simulink model "snap_sys_clk_feng"  (R2019a)
settings: Solver=VariableStepDiscrete  StartTime=0.0  StopTime=10.0  RelTol=1e-3
undefined symbols (not defined in the file): datetime, posixtime
libraries: xbsIndex_r4 x5252, casper_library_misc x69, xps_library x6, casper_library_delays x3
(part 5 of 45)

== system snap_sys_clk_feng/chan_reorder/skip_c_t_transpose ==
  sim_1 : Inport
  convert1_1 : DataTypeConversion  OutDataTypeStr=fixdt('ufix1_En0')  LockScale=on
  convert2_1 : DataTypeConversion  OutDataTypeStr=fixdt('ufix1_En0')  ConvertRealWorld=Stored Integer (SI)  LockScale=on
  gain_1 : Gain
  io_delay : xbsIndex_r4/Delay  rst=off  infoeditControl=Selection of Reset will increase slice count due to use of real FFs and instead of SRLs  en=off  latency=0  reg_retiming=on  dbl_ovrd=off  block_type=delay
  reint1 : xbsIndex_r4/Reinterpret  force_arith_type=on  arith_type=Unsigned  force_bin_pt=on  bin_pt=0  block_type=reinterpret
  slice_reg : xbsIndex_r4/Slice  nbits=1  boolean_output=off  mode=Lower Bit Location + Width  bit1=0  base1=MSB of Input  bit0=0  base0=LSB of Input  dbl_ovrd=off  block_type=slice
  snap_sys_clk_feng_chan_reorder_skip_c_t_transpose_user_data_out : xbsIndex_r4/Gateway In  gui_display_data_type=Fixed-point  arith_type=Unsigned  n_bits=32  bin_pt=0  preci_type=Single  exp_width=8  frac_width=24  rows=1  columns=1  quantization="Round  (unbiased: +/- Inf)"  overflow=Saturate  period=1  UseAsADC=off  ADCChannel='1'  interface=None  automatic_assignment=on  address_offset=hex2dec('00')  intf_name=''  intf_description=''  default_value=0  timing_constraint=None  locs_specified=off  LOCs={}  io_standard={}  inherit_from_input=off  hdl_port=on  dbl_ovrd=off  block_type=gatewayin
  in_reg : Outport
  wires:
  snap_sys_clk_feng_chan_reorder_skip_c_t_transpose_user_data_out/1 -> io_delay/1
  sim_1/1 -> convert1_1/1
  convert1_1/1 -> convert2_1/1
  convert2_1/1 -> gain_1/1
  gain_1/1 -> snap_sys_clk_feng_chan_reorder_skip_c_t_transpose_user_data_out/1
  io_delay/1 -> slice_reg/1
  slice_reg/1 -> reint1/1
  reint1/1 -> in_reg/1

== system snap_sys_clk_feng/chan_reorder/slice_duplicate ==
  sync : Inport
  din : Inport  Port=2
  gpu_order : Inport  Port=3
  Delay1 : xbsIndex_r4/Delay  rst=off  infoeditControl=Selection of Reset will increase slice count due to use of real FFs and instead of SRLs  en=off  latency=1  reg_retiming=off  dbl_ovrd=off  block_type=delay
  Delay2 : xbsIndex_r4/Delay  rst=off  infoeditControl=Selection of Reset will increase slice count due to use of real FFs and instead of SRLs  en=off  latency=3  reg_retiming=off  dbl_ovrd=off  block_type=delay
  Delay3 : xbsIndex_r4/Delay  rst=off  infoeditControl=Selection of Reset will increase slice count due to use of real FFs and instead of SRLs  en=off  latency=3  reg_retiming=off  dbl_ovrd=off  block_type=delay
  Mux2 : xbsIndex_r4/Mux  inputs=2  en=off  latency=1  precision=Full  arith_type=Unsigned  n_bits=16  bin_pt=14  quantization=Truncate  overflow=Wrap  dbl_ovrd=off  block_type=mux
  bus_convert1 : Subsystem  AncestorBlock=casper_library_bus/bus_convert  mask(bus_convert){n_bits_in=[8 8 8 8 8 8 8 8], bin_pt_in=7, cmplx=on, n_bits_out=4, bin_pt_out=3, quantization=0, overflow=0, csp_latency=0, of=off, misc=off}
      mask prompts: n_bits_in "input bit widths"; bin_pt_in "input binary points"; cmplx "input complex"; n_bits_out "output bit widths"; bin_pt_out "output binary points"; quantization "quantization strategy (Truncate=0, Round  (unbiased: +/- Inf)=1, Round (unbiased: Even Values)=2)"; overflow "overflow strategy (Wrap=0, Saturate=1, Flag as error=2)"; csp_latency "latency"; of "overflow indication"; misc "misc support"
      mask help: Convert components of busses
      mask init:
      | bus_convert_init(gcb, ...
      |     'n_bits_in', n_bits_in, ...
      |     'bin_pt_in', bin_pt_in, ...
      |     'cmplx', cmplx, ...
      |     'n_bits_out', n_bits_out, ...
      |     'bin_pt_out', bin_pt_out, ...
      |     'quantization', quantization, ...
      |     'overflow', overflow, ...
      |     'csp_latency', csp_latency, ...
      |     'misc', misc, ...
      |     'of', of);
  swizz : Subsystem
  sync_out : Outport
  dout0 : Outport  Port=2
  dout1 : Outport  Port=3
  wires:
  sync/1 -> Delay2/1, swizz/1(sync)
  bus_convert1/1(dout) -> dout1/1, dout0/1
  din/1 -> swizz/2(din), Delay3/1
  gpu_order/1 -> Mux2/1
  swizz/2(dout) -> Mux2/3
  Delay1/1 -> sync_out/1
  Delay2/1 -> Delay1/1
  Delay3/1 -> Mux2/2
  Mux2/1 -> bus_convert1/1(din)

== system snap_sys_clk_feng/chan_reorder/transpose_t_c ==
  note: output:
      | 1024 chans x 4 times x 4 chans x 4 times x 2 pols
  note: output:
      | 4096 chans x 4 times x 4 time (parallel) x 2 pols
  sync : Inport
  din : Inport  Port=2
  bypass : Inport  Port=3
  Constant2 : xbsIndex_r4/Constant  const=1.0  gui_display_data_type=Boolean  arith_type=Boolean  n_bits=16  bin_pt=14  preci_type=Single  exp_width=8  frac_width=24  explicit_period=on  period=1  equ=P=C  opselect=C  inp2=PCIN>>17  opr=+  inp1=P  carry=CIN  dbl_ovrd=off  block_type=constant
  Delay : xbsIndex_r4/Delay  rst=off  infoeditControl=Selection of Reset will increase slice count due to use of real FFs and instead of SRLs  en=off  latency=1  reg_retiming=off  dbl_ovrd=off  block_type=delay
  Delay1 : xbsIndex_r4/Delay  rst=off  infoeditControl=Selection of Reset will increase slice count due to use of real FFs and instead of SRLs  en=off  latency=1  reg_retiming=off  dbl_ovrd=off  block_type=delay
  Mux1 : xbsIndex_r4/Mux  inputs=2  en=off  latency=1  precision=Full  arith_type=Unsigned  n_bits=16  bin_pt=14  quantization=Truncate  overflow=Wrap  dbl_ovrd=off  block_type=mux
  Mux2 : xbsIndex_r4/Mux  inputs=2  en=off  latency=1  precision=Full  arith_type=Unsigned  n_bits=16  bin_pt=14  quantization=Truncate  overflow=Wrap  dbl_ovrd=off  block_type=mux
  bus_create3 : Subsystem  AncestorBlock=casper_library_flow_control/bus_create  mask(bus_create){inputNum=4}
      mask prompts: inputNum "Number of inputs:"
      mask init:
      | bus_create_init(gcb,...
      |     'inputNum', inputNum);
  bus_expand3 : Subsystem  AncestorBlock=casper_library_flow_control/bus_expand  mask(bus_expand){mode=divisions of equal size, outputNum=4, outputWidth=32, outputBinaryPt=0, outputArithmeticType=0, show_format=off, outputToWorkspace=off, variablePrefix=out, outputToModelAsWell=on}
      mask prompts: outputNum "Number of outputs:"; outputWidth "Output width:"; outputBinaryPt "Output binary point position:"; outputArithmeticType "Output arithmetic type (ufix=0, fix=1, bool=2):"; show_format "Print format string?"; outputToWorkspace "Output to workspace?"; variablePrefix "Variable name prefix:"; outputToModelAsWell "Output to model as well?"
      mask help:
      | Expands a 'bus' made using a bus_create or Xilinx
      | concat block.
      | The input will be divided into the specified number
      | of outputs with the specified arithmetic types.
      | Divisions are made from most significant bit.
      mask init: same as snap_sys_clk_feng/corr/bus_expand
      settings: AttributesFormatString=4 outputs
      mask TypeOptions mode: divisions of equal size | divisions of arbitrary size
      mask Callback mode: bus_expand_callback();
      mask Callback outputWidth: bus_expand_callback();
      mask Callback outputToWorkspace: bus_expand_callback();
  reorder5 : Subsystem  AncestorBlock=casper_library_reorder/reorder  mask(reorder){map=reshape(permute(reshape([0:16 - 1], 4, 4), [2,1]), 16, 1), n_bits=128, n_inputs=1, bram_latency=3, map_latency=3, fanout_latency=2, double_buffer=0, bram_map=off, software_controlled=off}
      mask prompts: map "Output Order:"; n_bits "Data width in"; n_inputs "Number of inputs"; bram_latency "BRAM Latency"; map_latency "Map Latency"; fanout_latency "Fanout latency"; double_buffer "Double Buffer"; bram_map "Use BlockRAM for Map"; software_controlled "Use runtime software control"
      mask init: same as snap_sys_clk_feng/chan_reorder/reorder3
      settings: AttributesFormatString=order=2
      mask Help: eval('xlWeb(''http://casper.berkeley.edu/wiki/Reorder'')')
  square_transposer : Subsystem  AncestorBlock=casper_library_reorder/square_transposer  mask(square_transposer){n_inputs=2, async=off}
      mask prompts: n_inputs "Number of inputs (2^?):"; async "Aynchronus operation"
      mask init:
      | square_transposer_init(gcb,...
      |     'n_inputs', n_inputs, ...
      |     'async', async);
      settings: AttributesFormatString=n_inputs=2
      mask Help: eval('xlWeb(''http://casper.berkeley.edu/wiki/Square_transposer'')')
  sync_out : Outport
  dout : Outport  Port=2
  wires:
  square_transposer/4(out2) -> bus_create3/3(in3)
  square_transposer/2(out0) -> bus_create3/1(in1)
  bus_expand3/1(msb_out4) -> square_transposer/2(in0)
  bus_create3/1(bus_out) -> reorder5/3(din0)
  Constant2/1 -> reorder5/2(en)
  bus_expand3/2(out3) -> square_transposer/3(in1)
  din/1 -> Mux2/3, bus_expand3/1(bus_in)
  reorder5/2(valid) -> ?
  square_transposer/1(sync_out) -> reorder5/1(sync)
  bus_expand3/3(out2) -> square_transposer/4(in2)
  square_transposer/3(out1) -> bus_create3/2(in2)
  square_transposer/5(out3) -> bus_create3/4(in4)
  bus_expand3/4(lsb_out1) -> square_transposer/5(in3)
  reorder5/1(sync_out) -> Mux1/2
  Mux1/1 -> sync_out/1
  reorder5/3(dout0) -> Mux2/2
  Mux2/1 -> dout/1
  sync/1 -> square_transposer/1(sync), Mux1/3
  bypass/1 -> Delay/1, Delay1/1
  Delay/1 -> Mux2/1
  Delay1/1 -> Mux1/1

== system snap_sys_clk_feng/chan_reorder/use_8bit ==
  sim_1 : Inport
  convert1_1 : DataTypeConversion  OutDataTypeStr=fixdt('ufix1_En0')  LockScale=on
  convert2_1 : DataTypeConversion  OutDataTypeStr=fixdt('ufix1_En0')  ConvertRealWorld=Stored Integer (SI)  LockScale=on
  gain_1 : Gain
  io_delay : xbsIndex_r4/Delay  rst=off  infoeditControl=Selection of Reset will increase slice count due to use of real FFs and instead of SRLs  en=off  latency=0  reg_retiming=on  dbl_ovrd=off  block_type=delay
  reint1 : xbsIndex_r4/Reinterpret  force_arith_type=on  arith_type=Unsigned  force_bin_pt=on  bin_pt=0  block_type=reinterpret
  slice_reg : xbsIndex_r4/Slice  nbits=1  boolean_output=off  mode=Lower Bit Location + Width  bit1=0  base1=MSB of Input  bit0=0  base0=LSB of Input  dbl_ovrd=off  block_type=slice
  snap_sys_clk_feng_chan_reorder_use_8bit_user_data_out : xbsIndex_r4/Gateway In  gui_display_data_type=Fixed-point  arith_type=Unsigned  n_bits=32  bin_pt=0  preci_type=Single  exp_width=8  frac_width=24  rows=1  columns=1  quantization="Round  (unbiased: +/- Inf)"  overflow=Saturate  period=1  UseAsADC=off  ADCChannel='1'  interface=None  automatic_assignment=on  address_offset=hex2dec('00')  intf_name=''  intf_description=''  default_value=0  timing_constraint=None  locs_specified=off  LOCs={}  io_standard={}  inherit_from_input=off  hdl_port=on  dbl_ovrd=off  block_type=gatewayin
  in_reg : Outport
  wires:
  snap_sys_clk_feng_chan_reorder_use_8bit_user_data_out/1 -> io_delay/1
  sim_1/1 -> convert1_1/1
  convert1_1/1 -> convert2_1/1
  convert2_1/1 -> gain_1/1
  gain_1/1 -> snap_sys_clk_feng_chan_reorder_use_8bit_user_data_out/1
  io_delay/1 -> slice_reg/1
  slice_reg/1 -> reint1/1
  reint1/1 -> in_reg/1

== system snap_sys_clk_feng/corr/bus_expand ==
  bus_in : Inport
  reinterpret1 : xbsIndex_r4/Reinterpret  force_arith_type=on  arith_type=Unsigned  force_bin_pt=on  bin_pt=0  block_type=reinterpret
  reinterpret2 : xbsIndex_r4/Reinterpret  force_arith_type=on  arith_type=Unsigned  force_bin_pt=on  bin_pt=0  block_type=reinterpret
  slice1 : xbsIndex_r4/Slice  nbits=200  boolean_output=off  mode=Upper Bit Location + Width  bit1=-200  base1=MSB of Input  bit0=0  base0=LSB of Input  dbl_ovrd=off  block_type=slice
  slice2 : xbsIndex_r4/Slice  nbits=200  boolean_output=off  mode=Upper Bit Location + Width  bit1=0  base1=MSB of Input  bit0=0  base0=LSB of Input  dbl_ovrd=off  block_type=slice
  msb_out2 : Outport
  lsb_out1 : Outport  Port=2
  wires:
  bus_in/1 -> slice2/1, slice1/1
  slice2/1 -> reinterpret2/1
  reinterpret2/1 -> msb_out2/1
  slice1/1 -> reinterpret1/1
  reinterpret1/1 -> lsb_out1/1

== system snap_sys_clk_feng/corr/bus_expand1 ==
  bus_in : Inport
  reinterpret{1..4} (4 alike) : xbsIndex_r4/Reinterpret  force_arith_type=on  arith_type="Signed  (2's comp)"  force_bin_pt=on  bin_pt=0  block_type=reinterpret
  slice1 : xbsIndex_r4/Slice  nbits=50  boolean_output=off  mode=Upper Bit Location + Width  bit1=-150  base1=MSB of Input  bit0=0  base0=LSB of Input  dbl_ovrd=off  block_type=slice
  slice2 : xbsIndex_r4/Slice  nbits=50  boolean_output=off  mode=Upper Bit Location + Width  bit1=-100  base1=MSB of Input  bit0=0  base0=LSB of Input  dbl_ovrd=off  block_type=slice
  slice3 : xbsIndex_r4/Slice  nbits=50  boolean_output=off  mode=Upper Bit Location + Width  bit1=-50  base1=MSB of Input  bit0=0  base0=LSB of Input  dbl_ovrd=off  block_type=slice
  slice4 : xbsIndex_r4/Slice  nbits=50  boolean_output=off  mode=Upper Bit Location + Width  bit1=0  base1=MSB of Input  bit0=0  base0=LSB of Input  dbl_ovrd=off  block_type=slice
  msb_out4 : Outport
  out3 : Outport  Port=2
  out2 : Outport  Port=3
  lsb_out1 : Outport  Port=4
  wires:
  bus_in/1 -> slice4/1, slice3/1, slice2/1, slice1/1
  slice4/1 -> reinterpret4/1
  reinterpret4/1 -> msb_out4/1
  slice3/1 -> reinterpret3/1
  reinterpret3/1 -> out3/1
  slice2/1 -> reinterpret2/1
  reinterpret2/1 -> out2/1
  slice1/1 -> reinterpret1/1
  reinterpret1/1 -> lsb_out1/1

== system snap_sys_clk_feng/corr/bus_expand2 ==
  bus_in : Inport
  reinterpret{1..4} (4 alike) : xbsIndex_r4/Reinterpret  force_arith_type=on  arith_type="Signed  (2's comp)"  force_bin_pt=on  bin_pt=0  block_type=reinterpret
  slice1 : xbsIndex_r4/Slice  nbits=50  boolean_output=off  mode=Upper Bit Location + Width  bit1=-150  base1=MSB of Input  bit0=0  base0=LSB of Input  dbl_ovrd=off  block_type=slice
  slice2 : xbsIndex_r4/Slice  nbits=50  boolean_output=off  mode=Upper Bit Location + Width  bit1=-100  base1=MSB of Input  bit0=0  base0=LSB of Input  dbl_ovrd=off  block_type=slice
  slice3 : xbsIndex_r4/Slice  nbits=50  boolean_output=off  mode=Upper Bit Location + Width  bit1=-50  base1=MSB of Input  bit0=0  base0=LSB of Input  dbl_ovrd=off  block_type=slice
  slice4 : xbsIndex_r4/Slice  nbits=50  boolean_output=off  mode=Upper Bit Location + Width  bit1=0  base1=MSB of Input  bit0=0  base0=LSB of Input  dbl_ovrd=off  block_type=slice
  msb_out4 : Outport
  out3 : Outport  Port=2
  out2 : Outport  Port=3
  lsb_out1 : Outport  Port=4
  wires:
  bus_in/1 -> slice4/1, slice3/1, slice2/1, slice1/1
  slice4/1 -> reinterpret4/1
  reinterpret4/1 -> msb_out4/1
  slice3/1 -> reinterpret3/1
  reinterpret3/1 -> out3/1
  slice2/1 -> reinterpret2/1
  reinterpret2/1 -> out2/1
  slice1/1 -> reinterpret1/1
  reinterpret1/1 -> lsb_out1/1

== system snap_sys_clk_feng/corr/bus_expand3 ==
  bus_in : Inport
  reinterpret{1..4} (4 alike) : xbsIndex_r4/Reinterpret  force_arith_type=on  arith_type="Signed  (2's comp)"  force_bin_pt=on  bin_pt=0  block_type=reinterpret
  slice1 : xbsIndex_r4/Slice  nbits=50  boolean_output=off  mode=Upper Bit Location + Width  bit1=-150  base1=MSB of Input  bit0=0  base0=LSB of Input  dbl_ovrd=off  block_type=slice
  slice2 : xbsIndex_r4/Slice  nbits=50  boolean_output=off  mode=Upper Bit Location + Width  bit1=-100  base1=MSB of Input  bit0=0  base0=LSB of Input  dbl_ovrd=off  block_type=slice
  slice3 : xbsIndex_r4/Slice  nbits=50  boolean_output=off  mode=Upper Bit Location + Width  bit1=-50  base1=MSB of Input  bit0=0  base0=LSB of Input  dbl_ovrd=off  block_type=slice
  slice4 : xbsIndex_r4/Slice  nbits=50  boolean_output=off  mode=Upper Bit Location + Width  bit1=0  base1=MSB of Input  bit0=0  base0=LSB of Input  dbl_ovrd=off  block_type=slice
  msb_out4 : Outport
  out3 : Outport  Port=2
  out2 : Outport  Port=3
  lsb_out1 : Outport  Port=4
  wires:
  bus_in/1 -> slice4/1, slice3/1, slice2/1, slice1/1
  slice4/1 -> reinterpret4/1
  reinterpret4/1 -> msb_out4/1
  slice3/1 -> reinterpret3/1
  reinterpret3/1 -> out3/1
  slice2/1 -> reinterpret2/1
  reinterpret2/1 -> out2/1
  slice1/1 -> reinterpret1/1
  reinterpret1/1 -> lsb_out1/1

== system snap_sys_clk_feng/corr/bus_expand4 ==
  bus_in : Inport
  reinterpret{1..4} (4 alike) : xbsIndex_r4/Reinterpret  force_arith_type=on  arith_type="Signed  (2's comp)"  force_bin_pt=on  bin_pt=0  block_type=reinterpret
  slice1 : xbsIndex_r4/Slice  nbits=50  boolean_output=off  mode=Upper Bit Location + Width  bit1=-150  base1=MSB of Input  bit0=0  base0=LSB of Input  dbl_ovrd=off  block_type=slice
  slice2 : xbsIndex_r4/Slice  nbits=50  boolean_output=off  mode=Upper Bit Location + Width  bit1=-100  base1=MSB of Input  bit0=0  base0=LSB of Input  dbl_ovrd=off  block_type=slice
  slice3 : xbsIndex_r4/Slice  nbits=50  boolean_output=off  mode=Upper Bit Location + Width  bit1=-50  base1=MSB of Input  bit0=0  base0=LSB of Input  dbl_ovrd=off  block_type=slice
  slice4 : xbsIndex_r4/Slice  nbits=50  boolean_output=off  mode=Upper Bit Location + Width  bit1=0  base1=MSB of Input  bit0=0  base0=LSB of Input  dbl_ovrd=off  block_type=slice
  msb_out4 : Outport
  out3 : Outport  Port=2
  out2 : Outport  Port=3
  lsb_out1 : Outport  Port=4
  wires:
  bus_in/1 -> slice4/1, slice3/1, slice2/1, slice1/1
  slice4/1 -> reinterpret4/1
  reinterpret4/1 -> msb_out4/1
  slice3/1 -> reinterpret3/1
  reinterpret3/1 -> out3/1
  slice2/1 -> reinterpret2/1
  reinterpret2/1 -> out2/1
  slice1/1 -> reinterpret1/1
  reinterpret1/1 -> lsb_out1/1

== system snap_sys_clk_feng/corr/crosspower_vacc ==
  new_acc : Inport
  x0 : Inport  Port=2
  x1 : Inport  Port=3
  x2 : Inport  Port=4
  x3 : Inport  Port=5
  y0 : Inport  Port=6
  y1 : Inport  Port=7
  y2 : Inport  Port=8
  y3 : Inport  Port=9
  Delay : xbsIndex_r4/Delay  rst=off  infoeditControl=Selection of Reset will increase slice count due to use of real FFs and instead of SRLs  en=off  latency=8  reg_retiming=off  dbl_ovrd=off  block_type=delay
  c_to_ri{,1..3} (4 alike) : casper_library_misc/c_to_ri  n_bits=bw+bw+1  bin_pt=bw-1 + bw-1
      settings: AttributesFormatString=51_48 r/i  SourceProductName=CASPER DSP Blockset
  cmult1 : Subsystem  AncestorBlock=casper_library_multipliers/cmult  mask(cmult){n_bits_a=25, bin_pt_a=24, n_bits_b=25, bin_pt_b=24, n_bits_ab=51, bin_pt_ab=48, quantization=Truncate, overflow=Wrap, conjugated=on, async=off, pipelined_enable=on, floating_point=off, float_type=single, exp_width=8, frac_width=24, in_latency=0, mult_latency=6, add_latency=2, conv_latency=0, pipeline_cmult_en=off, pipeline_latency=0, multiplier_implementation=behavioral HDL}
      mask prompts: n_bits_a "Number of Bits 'a'"; bin_pt_a "Binary Point 'a'"; n_bits_b "Number of Bits 'b'"; bin_pt_b "Binary Point 'b'"; n_bits_ab "Number of Bits 'ab'"; bin_pt_ab "Binary Point 'ab'"; conjugated "Conjugate"; async "asynchronous operation"; pipelined_enable "enable pipeline"; floating_point "floating point"; float_type "float type"; exp_width "exponent width"; frac_width "fraction width"; in_latency "Input latency"; mult_latency "Multiplier Latency"; add_latency "Adder Latency"; conv_latency "Convert latency"; pipeline_cmult_en "Pipeline cmult enable"; pipeline_latency "Pipeline latency"; multiplier_implementation "Multiplier implementation"
      mask help:
      | Multiplies two complex numbers using 4 multipliers and 2 adders.
      | Conjugation is optional.
      mask init:
      | cmult_init(gcb, ...
      |     'n_bits_a',n_bits_a, ...
      |     'bin_pt_a',bin_pt_a, ...
      |     'n_bits_b',n_bits_b, ...
      |     'bin_pt_b',bin_pt_b, ...
      |     'n_bits_ab',n_bits_ab, ...
      |     'bin_pt_ab',bin_pt_ab, ...
      |     'quantization',quantization, ...
      |     'floating_point', floating_point, ...
      |     'float_type', float_type, ...
      |     'exp_width', exp_width, ...
      |     'frac_width', frac_width, ...    
      |     'overflow', overflow, ...
      |     'in_latency', in_latency, ...
      |     'mult_latency', mult_latency, ...
      |     'add_latency', add_latency, ...
      |     'conv_latency', conv_latency, ...
      |     'conjugated', conjugated, ...
      |     'pipeline_cmult_en', pipeline_cmult_en, ...
      |     'pipeline_latency', pipeline_latency, ...
      |     'multiplier_implementation', multiplier_implementation, ...
      |     'async', async, ...
      |     'pipelined_enable', pipelined_enable);
      settings: AttributesFormatString=|
      | 25_24 * 25_24 ==> 51_48
      | Truncate, Wrap
      | Latency=0
      mask TypeOptions quantization: Truncate | Round  (unbiased: +/- Inf) | Round  (unbiased: Even Values)
      mask TypeOptions overflow: Wrap | Saturate | Flag as error
      mask Callback floating_point:
      | onoff = get_param(gcb, 'floating_point');
      | if strcmp(onoff,'on')
      |     enable_fixpt = 'off'
      |     set_param_state(gcb, 'float_type', 'on')
      | 
      |     f_type = get_param(gcb, 'float_type')
      |     if strcmp(f_type,'custom')
      |         set_param_state(gcb, 'exp_width', 'on')
      |         set_param_state(gcb, 'frac_width', 'on')
      |     else
      |         set_param_state(gcb, 'exp_width', 'off')
      |         set_param_state(gcb, 'frac_width', 'off')
      |     end
      | 
      | 
      | else
      |     enable_fixpt = 'on'
      |     set_param_state(gcb, 'float_type', 'off')
      |     set_param_state(gcb, 'exp_width', 'off')
      |     set_param_state(gcb, 'frac_width', 'off')
      | end
      | 
      | 
      | set_param_state(gcb, 'n_bits_a', enable_fixpt)
      | set_param_state(gcb, 'bin_pt_a', enable_fixpt)
      | set_param_state(gcb, 'n_bits_b', enable_fixpt)
      | set_param_state(gcb, 'bin_pt_b', enable_fixpt)
      | set_param_state(gcb, 'n_bits_ab', enable_fixpt)
      | set_param_state(gcb, 'bin_pt_ab', enable_fixpt)
      mask TypeOptions float_type: single | custom
      mask Callback float_type:
      | f_type = get_param(gcb, 'float_type')
      | if strcmp(f_type,'custom')
      |     set_param_state(gcb, 'exp_width', 'on')
      |     set_param_state(gcb, 'frac_width', 'on')
      | else
      |     set_param_state(gcb, 'exp_width', 'off')
      |     set_param_state(gcb, 'frac_width', 'off')
      | end
      mask Callback pipeline_cmult_en:
      | pipeline_en = get_param(gcb, 'pipeline_cmult_en');
      | if strcmp(pipeline_en,'on')
      | 
      |     set_param_state(gcb, 'pipeline_latency', 'on')
      | else
      |     set_param_state(gcb, 'pipeline_latency', 'off')
      | end
      mask TypeOptions multiplier_implementation: behavioral HDL | standard core | embedded multiplier core
      mask DialogControl ParameterTabVar0 Prompt: basic
      mask DialogControl ParameterTabVar01 Prompt: latency
      mask DialogControl ParameterTabVar012 Prompt: implementation
  cmult2 : Subsystem  AncestorBlock=casper_library_multipliers/cmult  mask(cmult){n_bits_a=25, bin_pt_a=24, n_bits_b=25, bin_pt_b=24, n_bits_ab=51, bin_pt_ab=48, quantization=Truncate, overflow=Wrap, conjugated=on, async=off, pipelined_enable=on, floating_point=off, float_type=single, exp_width=8, frac_width=24, in_latency=0, mult_latency=6, add_latency=2, conv_latency=0, pipeline_cmult_en=off, pipeline_latency=0, multiplier_implementation=behavioral HDL}
      mask prompts: n_bits_a "Number of Bits 'a'"; bin_pt_a "Binary Point 'a'"; n_bits_b "Number of Bits 'b'"; bin_pt_b "Binary Point 'b'"; n_bits_ab "Number of Bits 'ab'"; bin_pt_ab "Binary Point 'ab'"; conjugated "Conjugate"; async "asynchronous operation"; pipelined_enable "enable pipeline"; floating_point "floating point"; float_type "float type"; exp_width "exponent width"; frac_width "fraction width"; in_latency "Input latency"; mult_latency "Multiplier Latency"; add_latency "Adder Latency"; conv_latency "Convert latency"; pipeline_cmult_en "Pipeline cmult enable"; pipeline_latency "Pipeline latency"; multiplier_implementation "Multiplier implementation"
      mask help:
      | Multiplies two complex numbers using 4 multipliers and 2 adders.
      | Conjugation is optional.
      mask init: same as snap_sys_clk_feng/corr/crosspower_vacc/cmult1
      settings: AttributesFormatString=|
      | 25_24 * 25_24 ==> 51_48
      | Truncate, Wrap
      | Latency=0
      mask TypeOptions quantization: Truncate | Round  (unbiased: +/- Inf) | Round  (unbiased: Even Values)
      mask TypeOptions overflow: Wrap | Saturate | Flag as error
      mask Callback floating_point:
      | onoff = get_param(gcb, 'floating_point');
      | if strcmp(onoff,'on')
      |     enable_fixpt = 'off'
      |     set_param_state(gcb, 'float_type', 'on')
      | 
      |     f_type = get_param(gcb, 'float_type')
      |     if strcmp(f_type,'custom')
      |         set_param_state(gcb, 'exp_width', 'on')
      |         set_param_state(gcb, 'frac_width', 'on')
      |     else
      |         set_param_state(gcb, 'exp_width', 'off')
      |         set_param_state(gcb, 'frac_width', 'off')
      |     end
      | 
      | 
      | else
      |     enable_fixpt = 'on'
      |     set_param_state(gcb, 'float_type', 'off')
      |     set_param_state(gcb, 'exp_width', 'off')
      |     set_param_state(gcb, 'frac_width', 'off')
      | end
      | 
      | 
      | set_param_state(gcb, 'n_bits_a', enable_fixpt)
      | set_param_state(gcb, 'bin_pt_a', enable_fixpt)
      | set_param_state(gcb, 'n_bits_b', enable_fixpt)
      | set_param_state(gcb, 'bin_pt_b', enable_fixpt)
      | set_param_state(gcb, 'n_bits_ab', enable_fixpt)
      | set_param_state(gcb, 'bin_pt_ab', enable_fixpt)
      mask TypeOptions float_type: single | custom
      mask Callback float_type:
      | f_type = get_param(gcb, 'float_type')
      | if strcmp(f_type,'custom')
      |     set_param_state(gcb, 'exp_width', 'on')
      |     set_param_state(gcb, 'frac_width', 'on')
      | else
      |     set_param_state(gcb, 'exp_width', 'off')
      |     set_param_state(gcb, 'frac_width', 'off')
      | end
      mask Callback pipeline_cmult_en:
      | pipeline_en = get_param(gcb, 'pipeline_cmult_en');
      | if strcmp(pipeline_en,'on')
      | 
      |     set_param_state(gcb, 'pipeline_latency', 'on')
      | else
      |     set_param_state(gcb, 'pipeline_latency', 'off')
      | end
      mask TypeOptions multiplier_implementation: behavioral HDL | standard core | embedded multiplier core
      mask DialogControl ParameterTabVar0 Prompt: basic
      mask DialogControl ParameterTabVar01 Prompt: latency
      mask DialogControl ParameterTabVar012 Prompt: implementation
  cmult3 : Subsystem  AncestorBlock=casper_library_multipliers/cmult  mask(cmult){n_bits_a=25, bin_pt_a=24, n_bits_b=25, bin_pt_b=24, n_bits_ab=51, bin_pt_ab=48, quantization=Truncate, overflow=Wrap, conjugated=on, async=off, pipelined_enable=on, floating_point=off, float_type=single, exp_width=8, frac_width=24, in_latency=0, mult_latency=6, add_latency=2, conv_latency=0, pipeline_cmult_en=off, pipeline_latency=0, multiplier_implementation=behavioral HDL}
      mask prompts: n_bits_a "Number of Bits 'a'"; bin_pt_a "Binary Point 'a'"; n_bits_b "Number of Bits 'b'"; bin_pt_b "Binary Point 'b'"; n_bits_ab "Number of Bits 'ab'"; bin_pt_ab "Binary Point 'ab'"; conjugated "Conjugate"; async "asynchronous operation"; pipelined_enable "enable pipeline"; floating_point "floating point"; float_type "float type"; exp_width "exponent width"; frac_width "fraction width"; in_latency "Input latency"; mult_latency "Multiplier Latency"; add_latency "Adder Latency"; conv_latency "Convert latency"; pipeline_cmult_en "Pipeline cmult enable"; pipeline_latency "Pipeline latency"; multiplier_implementation "Multiplier implementation"
      mask help:
      | Multiplies two complex numbers using 4 multipliers and 2 adders.
      | Conjugation is optional.
      mask init: same as snap_sys_clk_feng/corr/crosspower_vacc/cmult1
      settings: AttributesFormatString=|
      | 25_24 * 25_24 ==> 51_48
      | Truncate, Wrap
      | Latency=0
      mask TypeOptions quantization: Truncate | Round  (unbiased: +/- Inf) | Round  (unbiased: Even Values)
      mask TypeOptions overflow: Wrap | Saturate | Flag as error
      mask Callback floating_point:
      | onoff = get_param(gcb, 'floating_point');
      | if strcmp(onoff,'on')
      |     enable_fixpt = 'off'
      |     set_param_state(gcb, 'float_type', 'on')
      | 
      |     f_type = get_param(gcb, 'float_type')
      |     if strcmp(f_type,'custom')
      |         set_param_state(gcb, 'exp_width', 'on')
      |         set_param_state(gcb, 'frac_width', 'on')
      |     else
      |         set_param_state(gcb, 'exp_width', 'off')
      |         set_param_state(gcb, 'frac_width', 'off')
      |     end
      | 
      | 
      | else
      |     enable_fixpt = 'on'
      |     set_param_state(gcb, 'float_type', 'off')
      |     set_param_state(gcb, 'exp_width', 'off')
      |     set_param_state(gcb, 'frac_width', 'off')
      | end
      | 
      | 
      | set_param_state(gcb, 'n_bits_a', enable_fixpt)
      | set_param_state(gcb, 'bin_pt_a', enable_fixpt)
      | set_param_state(gcb, 'n_bits_b', enable_fixpt)
      | set_param_state(gcb, 'bin_pt_b', enable_fixpt)
      | set_param_state(gcb, 'n_bits_ab', enable_fixpt)
      | set_param_state(gcb, 'bin_pt_ab', enable_fixpt)
      mask TypeOptions float_type: single | custom
      mask Callback float_type:
      | f_type = get_param(gcb, 'float_type')
      | if strcmp(f_type,'custom')
      |     set_param_state(gcb, 'exp_width', 'on')
      |     set_param_state(gcb, 'frac_width', 'on')
      | else
      |     set_param_state(gcb, 'exp_width', 'off')
      |     set_param_state(gcb, 'frac_width', 'off')
      | end
      mask Callback pipeline_cmult_en:
      | pipeline_en = get_param(gcb, 'pipeline_cmult_en');
      | if strcmp(pipeline_en,'on')
      | 
      |     set_param_state(gcb, 'pipeline_latency', 'on')
      | else
      |     set_param_state(gcb, 'pipeline_latency', 'off')
      | end
      mask TypeOptions multiplier_implementation: behavioral HDL | standard core | embedded multiplier core
      mask DialogControl ParameterTabVar0 Prompt: basic
      mask DialogControl ParameterTabVar01 Prompt: latency
      mask DialogControl ParameterTabVar012 Prompt: implementation
  cmult4 : Subsystem  AncestorBlock=casper_library_multipliers/cmult  mask(cmult){n_bits_a=25, bin_pt_a=24, n_bits_b=25, bin_pt_b=24, n_bits_ab=51, bin_pt_ab=48, quantization=Truncate, overflow=Wrap, conjugated=on, async=off, pipelined_enable=on, floating_point=off, float_type=single, exp_width=8, frac_width=24, in_latency=0, mult_latency=6, add_latency=2, conv_latency=0, pipeline_cmult_en=off, pipeline_latency=0, multiplier_implementation=behavioral HDL}
      mask prompts: n_bits_a "Number of Bits 'a'"; bin_pt_a "Binary Point 'a'"; n_bits_b "Number of Bits 'b'"; bin_pt_b "Binary Point 'b'"; n_bits_ab "Number of Bits 'ab'"; bin_pt_ab "Binary Point 'ab'"; conjugated "Conjugate"; async "asynchronous operation"; pipelined_enable "enable pipeline"; floating_point "floating point"; float_type "float type"; exp_width "exponent width"; frac_width "fraction width"; in_latency "Input latency"; mult_latency "Multiplier Latency"; add_latency "Adder Latency"; conv_latency "Convert latency"; pipeline_cmult_en "Pipeline cmult enable"; pipeline_latency "Pipeline latency"; multiplier_implementation "Multiplier implementation"
      mask help:
      | Multiplies two complex numbers using 4 multipliers and 2 adders.
      | Conjugation is optional.
      mask init: same as snap_sys_clk_feng/corr/crosspower_vacc/cmult1
      settings: AttributesFormatString=|
      | 25_24 * 25_24 ==> 51_48
      | Truncate, Wrap
      | Latency=0
      mask TypeOptions quantization: Truncate | Round  (unbiased: +/- Inf) | Round  (unbiased: Even Values)
      mask TypeOptions overflow: Wrap | Saturate | Flag as error
      mask Callback floating_point:
      | onoff = get_param(gcb, 'floating_point');
      | if strcmp(onoff,'on')
      |     enable_fixpt = 'off'
      |     set_param_state(gcb, 'float_type', 'on')
      | 
      |     f_type = get_param(gcb, 'float_type')
      |     if strcmp(f_type,'custom')
      |         set_param_state(gcb, 'exp_width', 'on')
      |         set_param_state(gcb, 'frac_width', 'on')
      |     else
      |         set_param_state(gcb, 'exp_width', 'off')
      |         set_param_state(gcb, 'frac_width', 'off')
      |     end
      | 
      | 
      | else
      |     enable_fixpt = 'on'
      |     set_param_state(gcb, 'float_type', 'off')
      |     set_param_state(gcb, 'exp_width', 'off')
      |     set_param_state(gcb, 'frac_width', 'off')
      | end
      | 
      | 
      | set_param_state(gcb, 'n_bits_a', enable_fixpt)
      | set_param_state(gcb, 'bin_pt_a', enable_fixpt)
      | set_param_state(gcb, 'n_bits_b', enable_fixpt)
      | set_param_state(gcb, 'bin_pt_b', enable_fixpt)
      | set_param_state(gcb, 'n_bits_ab', enable_fixpt)
      | set_param_state(gcb, 'bin_pt_ab', enable_fixpt)
      mask TypeOptions float_type: single | custom
      mask Callback float_type:
      | f_type = get_param(gcb, 'float_type')
      | if strcmp(f_type,'custom')
      |     set_param_state(gcb, 'exp_width', 'on')
      |     set_param_state(gcb, 'frac_width', 'on')
      | else
      |     set_param_state(gcb, 'exp_width', 'off')
      |     set_param_state(gcb, 'frac_width', 'off')
      | end
      mask Callback pipeline_cmult_en:
      | pipeline_en = get_param(gcb, 'pipeline_cmult_en');
      | if strcmp(pipeline_en,'on')
      | 
      |     set_param_state(gcb, 'pipeline_latency', 'on')
      | else
      |     set_param_state(gcb, 'pipeline_latency', 'off')
      | end
      mask TypeOptions multiplier_implementation: behavioral HDL | standard core | embedded multiplier core
      mask DialogControl ParameterTabVar0 Prompt: basic
      mask DialogControl ParameterTabVar01 Prompt: latency
      mask DialogControl ParameterTabVar012 Prompt: implementation
  ri_to_c{,1..3} (4 alike) : casper_library_misc/ri_to_c
      settings: SourceProductName=CASPER DSP Blockset
  simple_bram_vacc : Subsystem  AncestorBlock=casper_library_accumulators/simple_bram_vacc  mask(simple_bram_vacc){vec_len=nchan/4, arith_type=Signed, n_bits=vacc_bw, bin_pt=vacc_bp}
      mask prompts: vec_len "Vector length:"; arith_type "Output type:"; n_bits "Bit width (output):"; bin_pt "Binary point (output):"
      mask help: This simple vector accumulator is based on a shift register. It outputs its previous accumulated vector after a new_acc pulse is received.
      mask init:
      | simple_bram_vacc_init(gcb, ...
      |     'vec_len', vec_len, ...
      |     'arith_type', arith_type, ...
      |     'n_bits', n_bits, ...
      |     'bin_pt', bin_pt);
      mask TypeOptions arith_type: Signed | Unsigned
  simple_bram_vacc1 : Subsystem  AncestorBlock=casper_library_accumulators/simple_bram_vacc  mask(simple_bram_vacc){vec_len=nchan/4, arith_type=Signed, n_bits=vacc_bw, bin_pt=vacc_bp}
      mask prompts: vec_len "Vector length:"; arith_type "Output type:"; n_bits "Bit width (output):"; bin_pt "Binary point (output):"
      mask help: This simple vector accumulator is based on a shift register. It outputs its previous accumulated vector after a new_acc pulse is received.
      mask init:
      | simple_bram_vacc_init(gcb, ...
      |     'vec_len', vec_len, ...
      |     'arith_type', arith_type, ...
      |     'n_bits', n_bits, ...
      |     'bin_pt', bin_pt);
      mask TypeOptions arith_type: Signed | Unsigned
  simple_bram_vacc2 : Subsystem  AncestorBlock=casper_library_accumulators/simple_bram_vacc  mask(simple_bram_vacc){vec_len=nchan/4, arith_type=Signed, n_bits=vacc_bw, bin_pt=vacc_bp}
      mask prompts: vec_len "Vector length:"; arith_type "Output type:"; n_bits "Bit width (output):"; bin_pt "Binary point (output):"
      mask help: This simple vector accumulator is based on a shift register. It outputs its previous accumulated vector after a new_acc pulse is received.
      mask init:
      | simple_bram_vacc_init(gcb, ...
      |     'vec_len', vec_len, ...
      |     'arith_type', arith_type, ...
      |     'n_bits', n_bits, ...
      |     'bin_pt', bin_pt);
      mask TypeOptions arith_type: Signed | Unsigned
  simple_bram_vacc3 : Subsystem  AncestorBlock=casper_library_accumulators/simple_bram_vacc  mask(simple_bram_vacc){vec_len=nchan/4, arith_type=Signed, n_bits=vacc_bw, bin_pt=vacc_bp}
      mask prompts: vec_len "Vector length:"; arith_type "Output type:"; n_bits "Bit width (output):"; bin_pt "Binary point (output):"
      mask help: This simple vector accumulator is based on a shift register. It outputs its previous accumulated vector after a new_acc pulse is received.
      mask init:
      | simple_bram_vacc_init(gcb, ...
      |     'vec_len', vec_len, ...
      |     'arith_type', arith_type, ...
      |     'n_bits', n_bits, ...
      |     'bin_pt', bin_pt);
      mask TypeOptions arith_type: Signed | Unsigned
  simple_bram_vacc4 : Subsystem  AncestorBlock=casper_library_accumulators/simple_bram_vacc  mask(simple_bram_vacc){vec_len=nchan/4, arith_type=Signed, n_bits=vacc_bw, bin_pt=vacc_bp}
      mask prompts: vec_len "Vector length:"; arith_type "Output type:"; n_bits "Bit width (output):"; bin_pt "Binary point (output):"
      mask help: This simple vector accumulator is based on a shift register. It outputs its previous accumulated vector after a new_acc pulse is received.
      mask init:
      | simple_bram_vacc_init(gcb, ...
      |     'vec_len', vec_len, ...
      |     'arith_type', arith_type, ...
      |     'n_bits', n_bits, ...
      |     'bin_pt', bin_pt);
      mask TypeOptions arith_type: Signed | Unsigned
  simple_bram_vacc5 : Subsystem  AncestorBlock=casper_library_accumulators/simple_bram_vacc  mask(simple_bram_vacc){vec_len=nchan/4, arith_type=Signed, n_bits=vacc_bw, bin_pt=vacc_bp}
      mask prompts: vec_len "Vector length:"; arith_type "Output type:"; n_bits "Bit width (output):"; bin_pt "Binary point (output):"
      mask help: This simple vector accumulator is based on a shift register. It outputs its previous accumulated vector after a new_acc pulse is received.
      mask init:
      | simple_bram_vacc_init(gcb, ...
      |     'vec_len', vec_len, ...
      |     'arith_type', arith_type, ...
      |     'n_bits', n_bits, ...
      |     'bin_pt', bin_pt);
      mask TypeOptions arith_type: Signed | Unsigned
  simple_bram_vacc6 : Subsystem  AncestorBlock=casper_library_accumulators/simple_bram_vacc  mask(simple_bram_vacc){vec_len=nchan/4, arith_type=Signed, n_bits=vacc_bw, bin_pt=vacc_bp}
      mask prompts: vec_len "Vector length:"; arith_type "Output type:"; n_bits "Bit width (output):"; bin_pt "Binary point (output):"
      mask help: This simple vector accumulator is based on a shift register. It outputs its previous accumulated vector after a new_acc pulse is received.
      mask init:
      | simple_bram_vacc_init(gcb, ...
      |     'vec_len', vec_len, ...
      |     'arith_type', arith_type, ...
      |     'n_bits', n_bits, ...
      |     'bin_pt', bin_pt);
      mask TypeOptions arith_type: Signed | Unsigned
  simple_bram_vacc7 : Subsystem  AncestorBlock=casper_library_accumulators/simple_bram_vacc  mask(simple_bram_vacc){vec_len=nchan/4, arith_type=Signed, n_bits=vacc_bw, bin_pt=vacc_bp}
      mask prompts: vec_len "Vector length:"; arith_type "Output type:"; n_bits "Bit width (output):"; bin_pt "Binary point (output):"
      mask help: This simple vector accumulator is based on a shift register. It outputs its previous accumulated vector after a new_acc pulse is received.
      mask init:
      | simple_bram_vacc_init(gcb, ...
      |     'vec_len', vec_len, ...
      |     'arith_type', arith_type, ...
      |     'n_bits', n_bits, ...
      |     'bin_pt', bin_pt);
      mask TypeOptions arith_type: Signed | Unsigned
  vld : Outport
  xy0 : Outport  Port=2
  xy1 : Outport  Port=3
  xy2 : Outport  Port=4
  xy3 : Outport  Port=5
  wires:
  simple_bram_vacc/2(valid) -> vld/1
  x0/1 -> cmult4/1(a)
  new_acc/1 -> Delay/1
  x1/1 -> cmult1/1(a)
  y1/1 -> cmult1/2(b)
  y0/1 -> cmult4/2(b)
  cmult4/1(ab) -> c_to_ri/1
  cmult1/1(ab) -> c_to_ri1/1
  simple_bram_vacc/1(dout) -> ri_to_c/1
  simple_bram_vacc1/1(dout) -> ri_to_c/2
  ri_to_c/1 -> xy0/1
  simple_bram_vacc2/1(dout) -> ri_to_c1/1
  simple_bram_vacc3/1(dout) -> ri_to_c1/2
  ri_to_c1/1 -> xy1/1
  c_to_ri1/1 -> simple_bram_vacc2/2(din)
  c_to_ri1/2 -> simple_bram_vacc3/2(din)
  c_to_ri/2 -> simple_bram_vacc1/2(din)
  c_to_ri/1 -> simple_bram_vacc/2(din)
  Delay/1 -> simple_bram_vacc/1(new_acc), simple_bram_vacc1/1(new_acc), simple_bram_vacc2/1(new_acc), simple_bram_vacc3/1(new_acc), simple_bram_vacc4/1(new_acc), simple_bram_vacc5/1(new_acc), simple_bram_vacc7/1(new_acc), simple_bram_vacc6/1(new_acc)
  c_to_ri2/2 -> simple_bram_vacc5/2(din)
  c_to_ri3/2 -> simple_bram_vacc7/2(din)
  c_to_ri3/1 -> simple_bram_vacc6/2(din)
  ri_to_c3/1 -> xy3/1
  simple_bram_vacc7/1(dout) -> ri_to_c3/2
  simple_bram_vacc6/1(dout) -> ri_to_c3/1
  ri_to_c2/1 -> xy2/1
  simple_bram_vacc5/1(dout) -> ri_to_c2/2
  simple_bram_vacc4/1(dout) -> ri_to_c2/1
  cmult3/1(ab) -> c_to_ri3/1
  cmult2/1(ab) -> c_to_ri2/1
  y2/1 -> cmult2/2(b)
  y3/1 -> cmult3/2(b)
  x3/1 -> cmult3/1(a)
  x2/1 -> cmult2/1(a)
  simple_bram_vacc4/2(valid) -> ?
  c_to_ri2/1 -> simple_bram_vacc4/2(din)

== system snap_sys_clk_feng/corr/dest_ip ==
  sim_1 : Inport
  convert1_1 : DataTypeConversion  OutDataTypeStr=fixdt('ufix32_En0')  LockScale=on
  convert2_1 : DataTypeConversion  OutDataTypeStr=fixdt('ufix32_En0')  ConvertRealWorld=Stored Integer (SI)  LockScale=on
  gain_1 : Gain
  io_delay : xbsIndex_r4/Delay  rst=off  infoeditControl=Selection of Reset will increase slice count due to use of real FFs and instead of SRLs  en=off  latency=0  reg_retiming=on  dbl_ovrd=off  block_type=delay
  reint1 : xbsIndex_r4/Reinterpret  force_arith_type=on  arith_type=Unsigned  force_bin_pt=on  bin_pt=0  block_type=reinterpret
  slice_reg : xbsIndex_r4/Slice  nbits=32  boolean_output=off  mode=Lower Bit Location + Width  bit1=0  base1=MSB of Input  bit0=0  base0=LSB of Input  dbl_ovrd=off  block_type=slice
  snap_sys_clk_feng_corr_dest_ip_user_data_out : xbsIndex_r4/Gateway In  gui_display_data_type=Fixed-point  arith_type=Unsigned  n_bits=32  bin_pt=0  preci_type=Single  exp_width=8  frac_width=24  rows=1  columns=1  quantization="Round  (unbiased: +/- Inf)"  overflow=Saturate  period=1  UseAsADC=off  ADCChannel='1'  interface=None  automatic_assignment=on  address_offset=hex2dec('00')  intf_name=''  intf_description=''  default_value=0  timing_constraint=None  locs_specified=off  LOCs={}  io_standard={}  inherit_from_input=off  hdl_port=on  dbl_ovrd=off  block_type=gatewayin
  in_reg : Outport
  wires:
  snap_sys_clk_feng_corr_dest_ip_user_data_out/1 -> io_delay/1
  sim_1/1 -> convert1_1/1
  convert1_1/1 -> convert2_1/1
  convert2_1/1 -> gain_1/1
  gain_1/1 -> snap_sys_clk_feng_corr_dest_ip_user_data_out/1
  io_delay/1 -> slice_reg/1
  slice_reg/1 -> reint1/1
  reint1/1 -> in_reg/1

== system snap_sys_clk_feng/corr/feng_id ==
  sim_1 : Inport
  convert1_1 : DataTypeConversion  OutDataTypeStr=fixdt('ufix8_En0')  LockScale=on
  convert2_1 : DataTypeConversion  OutDataTypeStr=fixdt('ufix8_En0')  ConvertRealWorld=Stored Integer (SI)  LockScale=on
  gain_1 : Gain
  io_delay : xbsIndex_r4/Delay  rst=off  infoeditControl=Selection of Reset will increase slice count due to use of real FFs and instead of SRLs  en=off  latency=0  reg_retiming=on  dbl_ovrd=off  block_type=delay
  reint1 : xbsIndex_r4/Reinterpret  force_arith_type=on  arith_type=Unsigned  force_bin_pt=on  bin_pt=0  block_type=reinterpret
  slice_reg : xbsIndex_r4/Slice  nbits=8  boolean_output=off  mode=Lower Bit Location + Width  bit1=0  base1=MSB of Input  bit0=0  base0=LSB of Input  dbl_ovrd=off  block_type=slice
  snap_sys_clk_feng_corr_feng_id_user_data_out : xbsIndex_r4/Gateway In  gui_display_data_type=Fixed-point  arith_type=Unsigned  n_bits=32  bin_pt=0  preci_type=Single  exp_width=8  frac_width=24  rows=1  columns=1  quantization="Round  (unbiased: +/- Inf)"  overflow=Saturate  period=1  UseAsADC=off  ADCChannel='1'  interface=None  automatic_assignment=on  address_offset=hex2dec('00')  intf_name=''  intf_description=''  default_value=0  timing_constraint=None  locs_specified=off  LOCs={}  io_standard={}  inherit_from_input=off  hdl_port=on  dbl_ovrd=off  block_type=gatewayin
  in_reg : Outport
  wires:
  snap_sys_clk_feng_corr_feng_id_user_data_out/1 -> io_delay/1
  sim_1/1 -> convert1_1/1
  convert1_1/1 -> convert2_1/1
  convert2_1/1 -> gain_1/1
  gain_1/1 -> snap_sys_clk_feng_corr_feng_id_user_data_out/1
  io_delay/1 -> slice_reg/1
  slice_reg/1 -> reint1/1
  reint1/1 -> in_reg/1

== system snap_sys_clk_feng/corr/power_vacc0 ==
  new_acc : Inport
  in0 : Inport  Port=2
  in1 : Inport  Port=3
  in2 : Inport  Port=4
  in3 : Inport  Port=5
  Delay : xbsIndex_r4/Delay  rst=off  infoeditControl=Selection of Reset will increase slice count due to use of real FFs and instead of SRLs  en=off  latency=8  reg_retiming=off  dbl_ovrd=off  block_type=delay
  power{,1..3} (4 alike) : casper_library_misc/power  BitWidth=25  add_latency=2  mult_latency=6
      settings: SourceProductName=CASPER DSP Blockset
  simple_bram_vacc : Subsystem  AncestorBlock=casper_library_accumulators/simple_bram_vacc  mask(simple_bram_vacc){vec_len=nchan/4, arith_type=Signed, n_bits=vacc_bw, bin_pt=vacc_bp}
      mask prompts: vec_len "Vector length:"; arith_type "Output type:"; n_bits "Bit width (output):"; bin_pt "Binary point (output):"
      mask help: This simple vector accumulator is based on a shift register. It outputs its previous accumulated vector after a new_acc pulse is received.
      mask init:
      | simple_bram_vacc_init(gcb, ...
      |     'vec_len', vec_len, ...
      |     'arith_type', arith_type, ...
      |     'n_bits', n_bits, ...
      |     'bin_pt', bin_pt);
      mask TypeOptions arith_type: Signed | Unsigned
  simple_bram_vacc1 : Subsystem  AncestorBlock=casper_library_accumulators/simple_bram_vacc  mask(simple_bram_vacc){vec_len=nchan/4, arith_type=Signed, n_bits=vacc_bw, bin_pt=vacc_bp}
      mask prompts: vec_len "Vector length:"; arith_type "Output type:"; n_bits "Bit width (output):"; bin_pt "Binary point (output):"
      mask help: This simple vector accumulator is based on a shift register. It outputs its previous accumulated vector after a new_acc pulse is received.
      mask init:
      | simple_bram_vacc_init(gcb, ...
      |     'vec_len', vec_len, ...
      |     'arith_type', arith_type, ...
      |     'n_bits', n_bits, ...
      |     'bin_pt', bin_pt);
      mask TypeOptions arith_type: Signed | Unsigned
  simple_bram_vacc2 : Subsystem  AncestorBlock=casper_library_accumulators/simple_bram_vacc  mask(simple_bram_vacc){vec_len=nchan/4, arith_type=Signed, n_bits=vacc_bw, bin_pt=vacc_bp}
      mask prompts: vec_len "Vector length:"; arith_type "Output type:"; n_bits "Bit width (output):"; bin_pt "Binary point (output):"
      mask help: This simple vector accumulator is based on a shift register. It outputs its previous accumulated vector after a new_acc pulse is received.
      mask init:
      | simple_bram_vacc_init(gcb, ...
      |     'vec_len', vec_len, ...
      |     'arith_type', arith_type, ...
      |     'n_bits', n_bits, ...
      |     'bin_pt', bin_pt);
      mask TypeOptions arith_type: Signed | Unsigned
  simple_bram_vacc3 : Subsystem  AncestorBlock=casper_library_accumulators/simple_bram_vacc  mask(simple_bram_vacc){vec_len=nchan/4, arith_type=Signed, n_bits=vacc_bw, bin_pt=vacc_bp}
      mask prompts: vec_len "Vector length:"; arith_type "Output type:"; n_bits "Bit width (output):"; bin_pt "Binary point (output):"
      mask help: This simple vector accumulator is based on a shift register. It outputs its previous accumulated vector after a new_acc pulse is received.
      mask init:
      | simple_bram_vacc_init(gcb, ...
      |     'vec_len', vec_len, ...
      |     'arith_type', arith_type, ...
      |     'n_bits', n_bits, ...
      |     'bin_pt', bin_pt);
      mask TypeOptions arith_type: Signed | Unsigned
  vld : Outport
  out0 : Outport  Port=2
  out1 : Outport  Port=3
  out2 : Outport  Port=4
  out3 : Outport  Port=5
  wires:
  simple_bram_vacc1/1(dout) -> out1/1
  simple_bram_vacc/1(dout) -> out0/1
  in1/1 -> power1/1
  simple_bram_vacc/2(valid) -> vld/1
  in0/1 -> power/1
  new_acc/1 -> Delay/1
  Delay/1 -> simple_bram_vacc/1(new_acc), simple_bram_vacc2/1(new_acc), simple_bram_vacc3/1(new_acc), simple_bram_vacc1/1(new_acc)
  simple_bram_vacc2/1(dout) -> out2/1
  simple_bram_vacc3/1(dout) -> out3/1
  in2/1 -> power2/1
  in3/1 -> power3/1
  power/1 -> simple_bram_vacc/2(din)
  power1/1 -> simple_bram_vacc1/2(din)
  power2/1 -> simple_bram_vacc2/2(din)
  power3/1 -> simple_bram_vacc3/2(din)
